simulink model "M1_Solution_ComparePlants"  (R2026a)
settings: Solver=ode15s  StopTime=2  MaxStep=0.001
libraries: cstblocks_lti x1
settings Model: Creator=siddh  LastModifiedBy=sjawahar

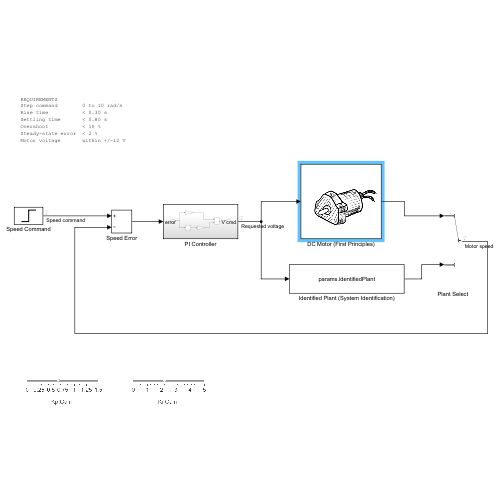
[thumbnail: Simulink's stored preview of the top-level diagram]
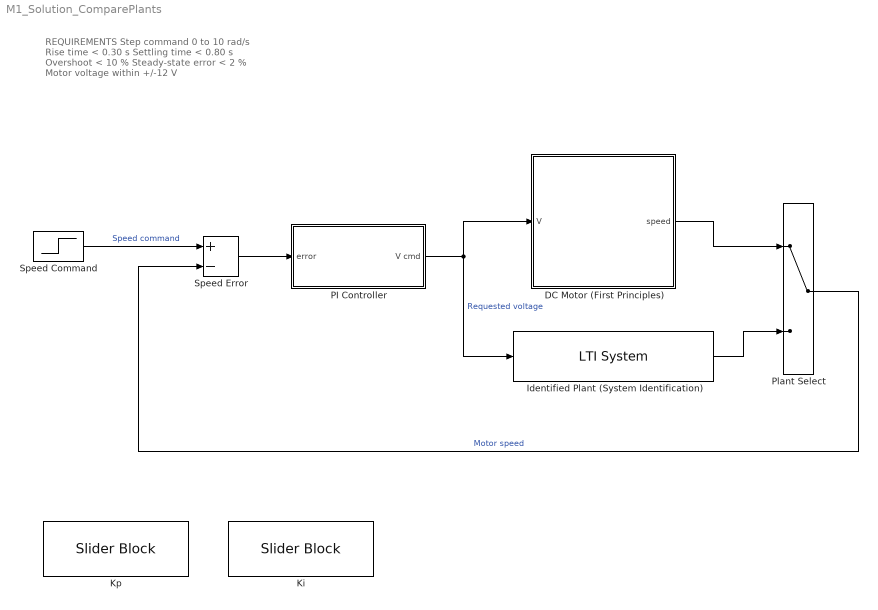
== system M1_Solution_ComparePlants ==
  note: REQUIREMENTS
      | Step command        0 to 10 rad/s
      | Rise time           < 0.30 s
      | Settling time       < 0.80 s
      | Overshoot           < 10 %
      | Steady-state error  < 2 %
      | Motor voltage       within +/-12 V
  DC Motor (First Principles) : Subsystem
      mask Display: image('DC motor.png')
  Identified Plant (System Identification) : cstblocks_lti/LTI System  sys=params.identifiedPlant  IC=[]  PadeOrder=0
      settings: LibrarySourceBlock=cstblocks/LTI System
  Ki : SliderBlock  LabelPosition=Bottom  ScaleMax=5
  Kp : SliderBlock  LabelPosition=Bottom  ScaleMax=1.5
  PI Controller : Subsystem
  Plant Select : ManualSwitch
  Speed Command : Step  Time=0.1  FinalValue=10  SampleTime=0
  Speed Error : Sum  Inputs=+-
  wires:
  Speed Command/1 -> Speed Error/1  "Speed command"
  Speed Error/1 -> PI Controller/1(error)
  PI Controller/1(V cmd) -> DC Motor (First Principles)/1(V), Identified Plant (System Identification)/1  "Requested voltage"
  DC Motor (First Principles)/1(speed) -> Plant Select/1
  Identified Plant (System Identification)/1 -> Plant Select/2
  Plant Select/1 -> Speed Error/2  "Motor speed"

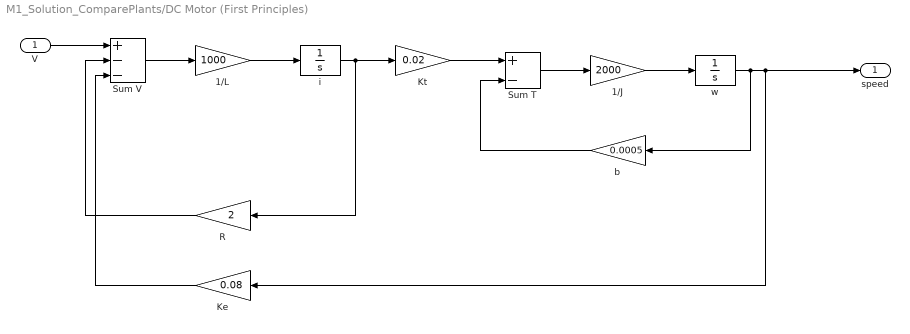
== system M1_Solution_ComparePlants/DC Motor (First Principles) ==
  V : Inport
  1/J : Gain  Gain=2000
  1/L : Gain  Gain=1000
  Ke : Gain  Gain=0.08
  Kt : Gain  Gain=0.02
  R : Gain  Gain=2
  Sum T : Sum  Inputs=+-
  Sum V : Sum  Inputs=+--
  b : Gain  Gain=0.0005
  i : Integrator
  w : Integrator
  speed : Outport
  wires:
  V/1 -> Sum V/1
  Sum V/1 -> 1/L/1
  1/L/1 -> i/1
  i/1 -> Kt/1, R/1
  Kt/1 -> Sum T/1
  Sum T/1 -> 1/J/1
  1/J/1 -> w/1
  w/1 -> speed/1, Ke/1, b/1
  b/1 -> Sum T/2
  R/1 -> Sum V/2
  Ke/1 -> Sum V/3

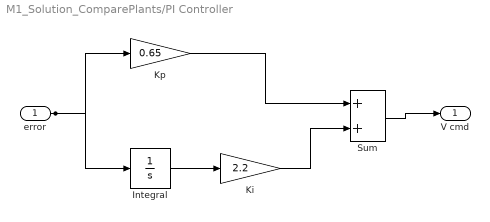
== system M1_Solution_ComparePlants/PI Controller ==
  error : Inport
  Integral : Integrator
  Ki : Gain  Gain=2.2
  Kp : Gain  Gain=0.65
  Sum : Sum
  V cmd : Outport
  wires:
  error/1 -> Kp/1, Integral/1
  Integral/1 -> Ki/1
  Kp/1 -> Sum/1
  Ki/1 -> Sum/2
  Sum/1 -> V cmd/1
